simulink model "ASM_Traffic_A11"  (R2026a)
settings: Solver=ode1  StartTime=SIM.tstart.v  StopTime=SIM.tend.v  FixedStep=SIM.StepSize.v
PostLoadFcn:
  | if any(exist('dsrtsu_mdlpostloadfcn', 'file') ~= 0), dsrtsu_mdlpostloadfcn('Execute', bdroot); end
  | try, asm_mdl_postloadfcn(bdroot, 'UpdateModel', 3600); catch, disp(lasterr); end,
InitFcn:
  | , if any(exist('rtifpga_mdlclblib', 'file') ~= 0), rtifpga_mdlclblib('Init', bdroot); end,
  | , if any(exist('dsmpb_private', 'file') ~= 0), dsmpb_private('dsmpb_mdlclblib', 'Init', bdroot); end,
undefined symbols (not defined in the file): _to_, a0b2, ASM_BrakeHydraulics_DemoSystems, ASM_VehicleDynamics_DemoSystems, b98103fe8ad365046cd0, BrakeCircuit, controllerConfig, CPT, Crankshaft, DiscIntNeverNeededParam, dsmsi, FinalDriveAssembly, instance, MDL, ModeSignals, mu, Pos_BrakePedal_Maneuver, rad, RefSignals, s_to_rpm, SIM, SoftECU, Suspension, Tire, Transmission
libraries: ASM_Traffic_lib x135, simulink x98, ASM_Utils_lib x77, ASM_VehicleDynamics_lib x70, ASM_Environment_lib x22, dsmpblib x20, dsmsilib x15, MDLD_Utils_lib x10, ASM_BrakeHydraulics_lib x3, sl_discontinuities x2
(part 29 of 63)

== system ASM_Traffic_A11/VehicleDynamics/Control/Sw_ECU_Brake_Signals/Enable_TrqDecrease_Fast_ESP[0|1] ==
  SoftECU : Inport
  RealECU : Inport  Port=2
  Const_Enable_TrqDecrease_Fast[0|1] : Constant  Value=0
  MultiPortSwitch : MultiPortSwitch
  Sw_Enable_TrqDecrease_Fast[1SoftECU|2RealECU|3Const] : Constant  Value=CPT.MDL_SW.Sw_Enable_TrqDecrease_Fast_ESP.v
  Enable_TrqDecrease_Fast[0|1] : Outport  VectorParamsAs1DForOutWhenUnconnected=off
  wires:
  Sw_Enable_TrqDecrease_Fast[1SoftECU|2RealECU|3Const]/1 -> MultiPortSwitch/1
  SoftECU/1 -> MultiPortSwitch/2
  RealECU/1 -> MultiPortSwitch/3
  Const_Enable_TrqDecrease_Fast[0|1]/1 -> MultiPortSwitch/4
  MultiPortSwitch/1 -> Enable_TrqDecrease_Fast[0|1]/1

== system ASM_Traffic_A11/VehicleDynamics/Control/Sw_ECU_Brake_Signals/Enable_TrqDecrease_Slow_ESP[0|1] ==
  SoftECU : Inport
  RealECU : Inport  Port=2
  Const_Enable_TrqDecrease_Slow[0|1] : Constant  Value=0
  MultiPortSwitch : MultiPortSwitch
  Sw_Enable_TrqDecrease_Slow[1SoftECU|2RealECU|3Const] : Constant  Value=CPT.MDL_SW.Sw_Enable_TrqDecrease_Slow_ESP.v
  Enable_TrqDecrease_Slow[0|1] : Outport  VectorParamsAs1DForOutWhenUnconnected=off
  wires:
  Sw_Enable_TrqDecrease_Slow[1SoftECU|2RealECU|3Const]/1 -> MultiPortSwitch/1
  SoftECU/1 -> MultiPortSwitch/2
  RealECU/1 -> MultiPortSwitch/3
  Const_Enable_TrqDecrease_Slow[0|1]/1 -> MultiPortSwitch/4
  MultiPortSwitch/1 -> Enable_TrqDecrease_Slow[0|1]/1

== system ASM_Traffic_A11/VehicleDynamics/Control/Sw_ECU_Brake_Signals/Enable_TrqIncrease_ESP[0|1] ==
  SoftECU : Inport
  RealECU : Inport  Port=2
  Const_Enable_TrqIncrease[0|1] : Constant  Value=0
  MultiPortSwitch : MultiPortSwitch
  Sw_Enable_TrqIncrease[1SoftECU|2RealECU|3Const] : Constant  Value=CPT.MDL_SW.Sw_Enable_TrqIncrease_ESP.v
  Enable_TrqIncrease[0|1] : Outport  VectorParamsAs1DForOutWhenUnconnected=off
  wires:
  Sw_Enable_TrqIncrease[1SoftECU|2RealECU|3Const]/1 -> MultiPortSwitch/1
  SoftECU/1 -> MultiPortSwitch/2
  RealECU/1 -> MultiPortSwitch/3
  Const_Enable_TrqIncrease[0|1]/1 -> MultiPortSwitch/4
  MultiPortSwitch/1 -> Enable_TrqIncrease[0|1]/1

== system ASM_Traffic_A11/VehicleDynamics/Control/Sw_ECU_Brake_Signals/Enable_p_Brake_Desired[0|1] ==
  SoftECU : Inport
  RealECU : Inport  Port=2
  Const_Enable_p_Brake_Desired[0|1] : Constant  Value=0
  MultiPortSwitch : MultiPortSwitch
  Sw_Enable_p_Brake_Desired[1SoftECU|2RealECU|3Const] : Constant  Value=CPT.MDL_SW.Sw_Enable_p_Brake_Desired.v
  Enable_p_Brake_Desired[0|1] : Outport  VectorParamsAs1DForOutWhenUnconnected=off
  wires:
  MultiPortSwitch/1 -> Enable_p_Brake_Desired[0|1]/1
  Const_Enable_p_Brake_Desired[0|1]/1 -> MultiPortSwitch/4
  RealECU/1 -> MultiPortSwitch/3
  SoftECU/1 -> MultiPortSwitch/2
  Sw_Enable_p_Brake_Desired[1SoftECU|2RealECU|3Const]/1 -> MultiPortSwitch/1

== system ASM_Traffic_A11/VehicleDynamics/Control/Sw_ECU_Brake_Signals/Trq_DecreaseRequest_Fast_ESP[Nm] ==
  SoftECU : Inport
  RealECU : Inport  Port=2
  Const_Trq_DecreaseRequest_Fast[Nm] : Constant  Value=0
  MultiPortSwitch : MultiPortSwitch
  Sw_Trq_DecreaseRequest_Fast[1SoftECU|2RealECU|3Const] : Constant  Value=CPT.MDL_SW.Sw_Trq_DecreaseRequest_Fast_ESP.v
  Trq_DecreaseRequest_Fast[Nm] : Outport  VectorParamsAs1DForOutWhenUnconnected=off
  wires:
  MultiPortSwitch/1 -> Trq_DecreaseRequest_Fast[Nm]/1
  Const_Trq_DecreaseRequest_Fast[Nm]/1 -> MultiPortSwitch/4
  RealECU/1 -> MultiPortSwitch/3
  SoftECU/1 -> MultiPortSwitch/2
  Sw_Trq_DecreaseRequest_Fast[1SoftECU|2RealECU|3Const]/1 -> MultiPortSwitch/1

== system ASM_Traffic_A11/VehicleDynamics/Control/Sw_ECU_Brake_Signals/Trq_DecreaseRequest_Slow_ESP[Nm] ==
  SoftECU : Inport
  RealECU : Inport  Port=2
  Const_Trq_DecreaseRequest_Slow[Nm] : Constant  Value=0
  MultiPortSwitch : MultiPortSwitch
  Sw_Trq_DecreaseRequest_Slow[1SoftECU|2RealECU|3Const] : Constant  Value=CPT.MDL_SW.Sw_Trq_DecreaseRequest_Slow_ESP.v
  Trq_DecreaseRequest_Slow[Nm] : Outport  VectorParamsAs1DForOutWhenUnconnected=off
  wires:
  MultiPortSwitch/1 -> Trq_DecreaseRequest_Slow[Nm]/1
  Const_Trq_DecreaseRequest_Slow[Nm]/1 -> MultiPortSwitch/4
  RealECU/1 -> MultiPortSwitch/3
  SoftECU/1 -> MultiPortSwitch/2
  Sw_Trq_DecreaseRequest_Slow[1SoftECU|2RealECU|3Const]/1 -> MultiPortSwitch/1

== system ASM_Traffic_A11/VehicleDynamics/Control/Sw_ECU_Brake_Signals/Trq_IncreaseRequest_ESP[Nm] ==
  SoftECU : Inport
  RealECU : Inport  Port=2
  Const_Trq_IncreaseRequest[Nm] : Constant  Value=0
  MultiPortSwitch : MultiPortSwitch
  Sw_Trq_IncreaseRequest[1SoftECU|2RealECU|3Const] : Constant  Value=CPT.MDL_SW.Sw_Trq_IncreaseRequest_ESP.v
  Trq_IncreaseRequest[Nm] : Outport  VectorParamsAs1DForOutWhenUnconnected=off
  wires:
  MultiPortSwitch/1 -> Trq_IncreaseRequest[Nm]/1
  Const_Trq_IncreaseRequest[Nm]/1 -> MultiPortSwitch/4
  RealECU/1 -> MultiPortSwitch/3
  SoftECU/1 -> MultiPortSwitch/2
  Sw_Trq_IncreaseRequest[1SoftECU|2RealECU|3Const]/1 -> MultiPortSwitch/1

== system ASM_Traffic_A11/VehicleDynamics/Control/Sw_ECU_Brake_Signals/p_Brake_Desired[bar] ==
  SoftECU : Inport
  RealECU : Inport  Port=2
  Const_p_Brake_Desired[bar] : Constant  Value=0
  MultiPortSwitch : MultiPortSwitch
  Sw_p_Brake_Desired[1SoftECU|2RealECU|3Const] : Constant  Value=CPT.MDL_SW.Sw_p_Brake_Desired.v
  p_Brake_Desired[bar] : Outport  VectorParamsAs1DForOutWhenUnconnected=off
  wires:
  Sw_p_Brake_Desired[1SoftECU|2RealECU|3Const]/1 -> MultiPortSwitch/1
  SoftECU/1 -> MultiPortSwitch/2
  RealECU/1 -> MultiPortSwitch/3
  Const_p_Brake_Desired[bar]/1 -> MultiPortSwitch/4
  MultiPortSwitch/1 -> p_Brake_Desired[bar]/1

== system ASM_Traffic_A11/VehicleDynamics/Control/Sw_ECU_Steering_Signals/Trq_PowerSteering[Nm] ==
  SoftECU : Inport
  RealECU : Inport  Port=2
  Const_Trq_PowerSteering[Nm] : Constant  Value=0
  MultiPortSwitch : MultiPortSwitch
  Sw_PowerSteering[1SoftECU|2RealECU|3Const] : Constant  Value=CPT.MDL_SW.Sw_PowerSteering.v
  Trq_PowerSteering[Nm] : Outport  VectorParamsAs1DForOutWhenUnconnected=off
  wires:
  MultiPortSwitch/1 -> Trq_PowerSteering[Nm]/1
  Const_Trq_PowerSteering[Nm]/1 -> MultiPortSwitch/4
  RealECU/1 -> MultiPortSwitch/3
  SoftECU/1 -> MultiPortSwitch/2
  Sw_PowerSteering[1SoftECU|2RealECU|3Const]/1 -> MultiPortSwitch/1

== system ASM_Traffic_A11/VehicleDynamics/Control/UserInterface/ASMSignalBus_Control ==
  In : Inport
  Terminator_1 : Terminator
  tag scope: ASMBUS_VehicleDynamics_Control=global
  wires:
  In/1 -> [ASMBUS_VehicleDynamics_Control]  "Control"
  [ASMBUS_VehicleDynamics_Control] -> Terminator_1/1

== system ASM_Traffic_A11/VehicleDynamics/Control/UserInterface/DISP_Control ==
  In : Inport
  ECU_Brake : Subsystem
  wires:
  In/1 -> ECU_Brake/1(In)

== system ASM_Traffic_A11/VehicleDynamics/Control/UserInterface/PAR_Control ==
  ECU_Brake : Subsystem
  Out : Outport  VectorParamsAs1DForOutWhenUnconnected=off
  wires:
  ECU_Brake/1(SoftECU_Brake) -> Out/1

== system ASM_Traffic_A11/VehicleDynamics/Interface_In/ExternalSignals/ExternalECU_Brake ==
  Enable_p_Brake_Desired[0|1] : Inport
  p_Brake_Desired[bar] : Inport  Port=2
  Enable_TrqDecrease_Fast_ESP[0|1] : Inport  Port=3
  Trq_DecreaseRequest_Fast_ESP[Nm] : Inport  Port=4
  Enable_TrqDecrease_Slow_ESP[0|1] : Inport  Port=5
  Trq_DecreaseRequest_Slow_ESP[Nm] : Inport  Port=6
  Enable_TrqIncrease_ESP[0|1] : Inport  Port=7
  Trq_IncreaseRequest_ESP[Nm] : Inport  Port=8
  ECU_ESP_Mode[0None|1ABS|2ESP|3ASR] : Inport  Port=9
  Ctrl_InletValve_FL[0_1] : Inport  Port=10
  Ctrl_InletValve_FR[0_1] : Inport  Port=11
  Ctrl_InletValve_RL[0_1] : Inport  Port=12
  Ctrl_InletValve_RR[0_1] : Inport  Port=13
  Ctrl_OutletValve_FL[0_1] : Inport  Port=14
  Ctrl_OutletValve_FR[0_1] : Inport  Port=15
  Ctrl_OutletValve_RL[0_1] : Inport  Port=16
  Ctrl_OutletValve_RR[0_1] : Inport  Port=17
  Ctrl_PreChargeValve_1[0_1] : Inport  Port=18
  Ctrl_PreChargeValve_2[0_1] : Inport  Port=19
  Ctrl_ChangeOverValve_1[0_1] : Inport  Port=20
  Ctrl_ChangeOverValve_2[0_1] : Inport  Port=21
  Ctrl_HydPump[0_1] : Inport  Port=22
  Bus Creator2 : BusCreator  Inputs=22
  Out : Outport  VectorParamsAs1DForOutWhenUnconnected=off
  wires:
  Ctrl_InletValve_FL[0_1]/1 -> Bus Creator2/10  "Ctrl_InletValve_FL[0_1]"
  Bus Creator2/1 -> Out/1  "Brake"
  Ctrl_InletValve_FR[0_1]/1 -> Bus Creator2/11  "Ctrl_InletValve_FR[0_1]"
  Ctrl_InletValve_RL[0_1]/1 -> Bus Creator2/12  "Ctrl_InletValve_RL[0_1]"
  Ctrl_InletValve_RR[0_1]/1 -> Bus Creator2/13  "Ctrl_InletValve_RR[0_1]"
  Ctrl_OutletValve_FL[0_1]/1 -> Bus Creator2/14  "Ctrl_OutletValve_FL[0_1]"
  Ctrl_OutletValve_FR[0_1]/1 -> Bus Creator2/15  "Ctrl_OutletValve_FR[0_1]"
  Ctrl_OutletValve_RL[0_1]/1 -> Bus Creator2/16  "Ctrl_OutletValve_RL[0_1]"
  Ctrl_OutletValve_RR[0_1]/1 -> Bus Creator2/17  "Ctrl_OutletValve_RR[0_1]"
  Ctrl_PreChargeValve_1[0_1]/1 -> Bus Creator2/18  "Ctrl_PreChargeValve_1[0_1]"
  Ctrl_PreChargeValve_2[0_1]/1 -> Bus Creator2/19  "Ctrl_PreChargeValve_2[0_1]"
  Ctrl_ChangeOverValve_1[0_1]/1 -> Bus Creator2/20  "Ctrl_ChangeOverValve_1[0_1]"
  Ctrl_ChangeOverValve_2[0_1]/1 -> Bus Creator2/21  "Ctrl_ChangeOverValve_2[0_1]"
  Ctrl_HydPump[0_1]/1 -> Bus Creator2/22  "Ctrl_HydPump[0_1]"
  Enable_TrqDecrease_Fast_ESP[0|1]/1 -> Bus Creator2/3  "Enable_TrqDecrease_Fast_ESP[0|1]"
  Trq_DecreaseRequest_Slow_ESP[Nm]/1 -> Bus Creator2/6  "Trq_DecreaseRequest_Slow_ESP[Nm]"
  Enable_TrqIncrease_ESP[0|1]/1 -> Bus Creator2/7  "Enable_TrqIncrease_ESP[0|1]"
  Trq_IncreaseRequest_ESP[Nm]/1 -> Bus Creator2/8  "Trq_IncreaseRequest_ESP[Nm]"
  Trq_DecreaseRequest_Fast_ESP[Nm]/1 -> Bus Creator2/4  "Trq_DecreaseRequest_Fast_ESP[Nm]"
  Enable_TrqDecrease_Slow_ESP[0|1]/1 -> Bus Creator2/5  "Enable_TrqDecrease_Slow_ESP[0|1]"
  Enable_p_Brake_Desired[0|1]/1 -> Bus Creator2/1  "Enable_p_Brake_Desired[0|1]"
  p_Brake_Desired[bar]/1 -> Bus Creator2/2  "p_Brake_Desired[bar]"
  ECU_ESP_Mode[0None|1ABS|2ESP|3ASR]/1 -> Bus Creator2/9  "ECU_ESP_Mode[0None|1ABS|2ESP|3ASR]"

== system ASM_Traffic_A11/VehicleDynamics/Interface_In/ExternalSignals/ExternalECU_Steering ==
  Trq_PowerSteering[Nm] : Inport
  Bus Creator6 : BusCreator  Inputs=1
  Out : Outport  VectorParamsAs1DForOutWhenUnconnected=off
  wires:
  Bus Creator6/1 -> Out/1  "Steering"
  Trq_PowerSteering[Nm]/1 -> Bus Creator6/1  "Trq_PowerSteering[Nm]"

== system ASM_Traffic_A11/VehicleDynamics/Interface_In/ExternalSignals/ExternalPlant_EPSMotor ==
  Angle_EPSMotor[rad] : Inport
  Angle_dt_EPSMotor[rad|s] : Inport  Port=2
  Bus Creator6 : BusCreator  Inputs=2
  Out : Outport  VectorParamsAs1DForOutWhenUnconnected=off
  wires:
  Angle_dt_EPSMotor[rad|s]/1 -> Bus Creator6/2  "Angle_dt_EPSMotor[rad|s]"
  Bus Creator6/1 -> Out/1  "EPSMotor"
  Angle_EPSMotor[rad]/1 -> Bus Creator6/1  "Angle_EPSMotor[rad]"

== system ASM_Traffic_A11/VehicleDynamics/Interface_In/ExternalSignals/ExternalPlant_RollerDyno ==
  Angle_Gamma_FL_Wheel[deg] : Inport
  omega_Wheel[FL;FR;RL;RR][rad|s] : Inport  Port=2
  Bus Creator6 : BusCreator  Inputs=2
  Out : Outport  VectorParamsAs1DForOutWhenUnconnected=off
  wires:
  Angle_Gamma_FL_Wheel[deg]/1 -> Bus Creator6/1  "Angle_Gamma_FL_Wheel[deg]"
  omega_Wheel[FL;FR;RL;RR][rad|s]/1 -> Bus Creator6/2  "omega_Wheel[FL;FR;RL;RR][rad|s]"
  Bus Creator6/1 -> Out/1  "RollerDyno"

== system ASM_Traffic_A11/VehicleDynamics/Interface_In/ExternalSignals/ExternalPlant_Steering ==
  Displ_Steering[m] : Inport
  Displ_Steering_dt[m|s] : Inport  Port=2
  Bus Creator6 : BusCreator  Inputs=2
  Out : Outport  VectorParamsAs1DForOutWhenUnconnected=off
  wires:
  Displ_Steering_dt[m|s]/1 -> Bus Creator6/2  "Displ_Steering_dt[m|s]"
  Displ_Steering[m]/1 -> Bus Creator6/1  "Displ_Steering[m]"
  Bus Creator6/1 -> Out/1  "Steering"

== system ASM_Traffic_A11/VehicleDynamics/Interface_In/ModelSignals/Angle_SteeringWheel[deg]_ ==
  In1 : Inport
  Gain : Gain  SaturateOnIntegerOverflow=on  OutDataTypeStr=Inherit: Same as input  ParamDataTypeStr=Inherit: Same as input
  Out1 : Outport  VectorParamsAs1DForOutWhenUnconnected=off
  wires:
  In1/1 -> Gain/1
  Gain/1 -> Out1/1

== system ASM_Traffic_A11/VehicleDynamics/Interface_In/ModelSignals/Angle_Vehicle_Init_CoorSys_E[x;y;z][rad]_ ==
  In1 : Inport
  Gain : Gain  SaturateOnIntegerOverflow=on  OutDataTypeStr=Inherit: Same as input  ParamDataTypeStr=Inherit: Same as input
  Out1 : Outport  VectorParamsAs1DForOutWhenUnconnected=off
  wires:
  In1/1 -> Gain/1
  Gain/1 -> Out1/1

== system ASM_Traffic_A11/VehicleDynamics/Interface_In/ModelSignals/Const_Steering_Mode_Manual[1Angle|2Trq]_ ==
  In1 : Inport
  Gain : Gain  SaturateOnIntegerOverflow=on  OutDataTypeStr=Inherit: Same as input  ParamDataTypeStr=Inherit: Same as input
  Out1 : Outport  VectorParamsAs1DForOutWhenUnconnected=off
  wires:
  Gain/1 -> Out1/1
  In1/1 -> Gain/1

== system ASM_Traffic_A11/VehicleDynamics/Interface_In/ModelSignals/ECU_Commands[]_ ==
  In1 : Inport
  Gain : Gain  SaturateOnIntegerOverflow=on  OutDataTypeStr=Inherit: Same as input  ParamDataTypeStr=Inherit: Same as input
  Out1 : Outport  VectorParamsAs1DForOutWhenUnconnected=off
  wires:
  In1/1 -> Gain/1
  Gain/1 -> Out1/1

== system ASM_Traffic_A11/VehicleDynamics/Interface_In/ModelSignals/Enable_Trq_Brake_Extern[0|1]_ ==
  In1 : Inport
  Gain : Gain  SaturateOnIntegerOverflow=on  OutDataTypeStr=Inherit: Same as input  ParamDataTypeStr=Inherit: Same as input
  Out1 : Outport  VectorParamsAs1DForOutWhenUnconnected=off
  wires:
  In1/1 -> Gain/1
  Gain/1 -> Out1/1

== system ASM_Traffic_A11/VehicleDynamics/Interface_In/ModelSignals/Fric_Coeff_CP[FL;FR;RL;RR][]_ ==
  In1 : Inport
  Gain : Gain  SaturateOnIntegerOverflow=on  OutDataTypeStr=Inherit: Same as input  ParamDataTypeStr=Inherit: Same as input
  Out1 : Outport  VectorParamsAs1DForOutWhenUnconnected=off
  wires:
  In1/1 -> Gain/1
  Gain/1 -> Out1/1

== system ASM_Traffic_A11/VehicleDynamics/Interface_In/ModelSignals/Keep_VehiclePosition[0|1]_ ==
  In1 : Inport
  Gain : Gain  SaturateOnIntegerOverflow=on  OutDataTypeStr=Inherit: Same as input  ParamDataTypeStr=Inherit: Same as input
  Out1 : Outport  VectorParamsAs1DForOutWhenUnconnected=off
  wires:
  In1/1 -> Gain/1
  Gain/1 -> Out1/1

== system ASM_Traffic_A11/VehicleDynamics/Interface_In/ModelSignals/M_Articulated_T[1x36]_ ==
  In1 : Inport
  Gain : Gain  SaturateOnIntegerOverflow=on  OutDataTypeStr=Inherit: Same as input  ParamDataTypeStr=Inherit: Same as input
  Out1 : Outport  VectorParamsAs1DForOutWhenUnconnected=off
  wires:
  In1/1 -> Gain/1
  Gain/1 -> Out1/1

== system ASM_Traffic_A11/VehicleDynamics/Interface_In/ModelSignals/Pos_AccPedal[%]_ ==
  In1 : Inport
  Gain : Gain  SaturateOnIntegerOverflow=on  OutDataTypeStr=Inherit: Same as input  ParamDataTypeStr=Inherit: Same as input
  Out1 : Outport  VectorParamsAs1DForOutWhenUnconnected=off
  wires:
  In1/1 -> Gain/1
  Gain/1 -> Out1/1

== system ASM_Traffic_A11/VehicleDynamics/Interface_In/ModelSignals/Pos_BrakePedal[%]_ ==
  In1 : Inport
  Gain : Gain  SaturateOnIntegerOverflow=on  OutDataTypeStr=Inherit: Same as input  ParamDataTypeStr=Inherit: Same as input
  Out1 : Outport  VectorParamsAs1DForOutWhenUnconnected=off
  wires:
  In1/1 -> Gain/1
  Gain/1 -> Out1/1

== system ASM_Traffic_A11/VehicleDynamics/Interface_In/ModelSignals/Pos_Vehicle_Init_CoorSys_E[x;y;z][m]_ ==
  In1 : Inport
  Gain : Gain  SaturateOnIntegerOverflow=on  OutDataTypeStr=Inherit: Same as input  ParamDataTypeStr=Inherit: Same as input
  Out1 : Outport  VectorParamsAs1DForOutWhenUnconnected=off
  wires:
  In1/1 -> Gain/1
  Gain/1 -> Out1/1

== system ASM_Traffic_A11/VehicleDynamics/Interface_In/ModelSignals/Pos_z_CP[FL;FR;RL;RR][m]_ ==
  In1 : Inport
  Gain : Gain  SaturateOnIntegerOverflow=on  OutDataTypeStr=Inherit: Same as input  ParamDataTypeStr=Inherit: Same as input
  Out1 : Outport  VectorParamsAs1DForOutWhenUnconnected=off
  wires:
  In1/1 -> Gain/1
  Gain/1 -> Out1/1

== system ASM_Traffic_A11/VehicleDynamics/Interface_In/ModelSignals/Q_Articulated_T[6x1]_ ==
  In1 : Inport
  Gain : Gain  SaturateOnIntegerOverflow=on  OutDataTypeStr=Inherit: Same as input  ParamDataTypeStr=Inherit: Same as input
  Out1 : Outport  VectorParamsAs1DForOutWhenUnconnected=off
  wires:
  In1/1 -> Gain/1
  Gain/1 -> Out1/1

== system ASM_Traffic_A11/VehicleDynamics/Interface_In/ModelSignals/Reset_VehicleStates[0|1]_ ==
  In1 : Inport
  Gain : Gain  SaturateOnIntegerOverflow=on  OutDataTypeStr=Inherit: Same as input  ParamDataTypeStr=Inherit: Same as input
  Out1 : Outport  VectorParamsAs1DForOutWhenUnconnected=off
  wires:
  In1/1 -> Gain/1
  Gain/1 -> Out1/1

== system ASM_Traffic_A11/VehicleDynamics/Interface_In/ModelSignals/Sw_Ignition[0Off|1On]_ ==
  In1 : Inport
  Gain : Gain  SaturateOnIntegerOverflow=on  OutDataTypeStr=Inherit: Same as input  ParamDataTypeStr=Inherit: Same as input
  Out1 : Outport  VectorParamsAs1DForOutWhenUnconnected=off
  wires:
  In1/1 -> Gain/1
  Gain/1 -> Out1/1

== system ASM_Traffic_A11/VehicleDynamics/Interface_In/ModelSignals/Sw_ModelDeskPlottingInterface[0Disabled|1Enabled]_ ==
  In1 : Inport
  Gain : Gain
  Out1 : Outport
  wires:
  Gain/1 -> Out1/1
  In1/1 -> Gain/1

== system ASM_Traffic_A11/VehicleDynamics/Interface_In/ModelSignals/Sw_ModelPortBlocks[0Disabled|1Enabled]_ ==
  In1 : Inport
  Gain : Gain
  Out1 : Outport
  wires:
  Gain/1 -> Out1/1
  In1/1 -> Gain/1

== system ASM_Traffic_A11/VehicleDynamics/Interface_In/ModelSignals/Sw_ParkingBrake[0Off|1On]_ ==
  In1 : Inport
  Gain : Gain  SaturateOnIntegerOverflow=on  OutDataTypeStr=Inherit: Same as input  ParamDataTypeStr=Inherit: Same as input
  Out1 : Outport  VectorParamsAs1DForOutWhenUnconnected=off
  wires:
  In1/1 -> Gain/1
  Gain/1 -> Out1/1

== system ASM_Traffic_A11/VehicleDynamics/Interface_In/ModelSignals/Sw_SteeringMode[1Angle|2Trq]_ ==
  In1 : Inport
  Gain : Gain  SaturateOnIntegerOverflow=on  OutDataTypeStr=Inherit: Same as input  ParamDataTypeStr=Inherit: Same as input
  Out1 : Outport  VectorParamsAs1DForOutWhenUnconnected=off
  wires:
  In1/1 -> Gain/1
  Gain/1 -> Out1/1

== system ASM_Traffic_A11/VehicleDynamics/Interface_In/ModelSignals/Sw_Steering_Mode[1Manual|2ManSched]_ ==
  In1 : Inport
  Gain : Gain  SaturateOnIntegerOverflow=on  OutDataTypeStr=Inherit: Same as input  ParamDataTypeStr=Inherit: Same as input
  Out1 : Outport  VectorParamsAs1DForOutWhenUnconnected=off
  wires:
  Gain/1 -> Out1/1
  In1/1 -> Gain/1

== system ASM_Traffic_A11/VehicleDynamics/Interface_In/ModelSignals/Sw_Tire_Parameter_Set_CP[FL;FR;RL;RR][1|2|3|4]_ ==
  In1 : Inport
  Gain : Gain  SaturateOnIntegerOverflow=on  OutDataTypeStr=Inherit: Same as input  ParamDataTypeStr=Inherit: Same as input
  Out1 : Outport  VectorParamsAs1DForOutWhenUnconnected=off
  wires:
  In1/1 -> Gain/1
  Gain/1 -> Out1/1

== system ASM_Traffic_A11/VehicleDynamics/Interface_In/ModelSignals/T_Ambient[degC]_ ==
  In1 : Inport
  Gain : Gain  SaturateOnIntegerOverflow=on  OutDataTypeStr=Inherit: Same as input  ParamDataTypeStr=Inherit: Same as input
  Out1 : Outport  VectorParamsAs1DForOutWhenUnconnected=off
  wires:
  In1/1 -> Gain/1
  Gain/1 -> Out1/1

== system ASM_Traffic_A11/VehicleDynamics/Interface_In/ModelSignals/Trq_Brake_Request_Extern[Nm]_ ==
  In1 : Inport
  Gain : Gain  SaturateOnIntegerOverflow=on  OutDataTypeStr=Inherit: Same as input  ParamDataTypeStr=Inherit: Same as input
  Out1 : Outport  VectorParamsAs1DForOutWhenUnconnected=off
  wires:
  In1/1 -> Gain/1
  Gain/1 -> Out1/1

== system ASM_Traffic_A11/VehicleDynamics/Interface_In/ModelSignals/Trq_Driver_External[Nm]_ ==
  In1 : Inport
  Gain : Gain  SaturateOnIntegerOverflow=on  OutDataTypeStr=Inherit: Same as input  ParamDataTypeStr=Inherit: Same as input
  Out1 : Outport  VectorParamsAs1DForOutWhenUnconnected=off
  wires:
  In1/1 -> Gain/1
  Gain/1 -> Out1/1

== system ASM_Traffic_A11/VehicleDynamics/Interface_In/ModelSignals/Trq_EM_Front[Nm]_ ==
  In1 : Inport
  Gain : Gain  SaturateOnIntegerOverflow=on  OutDataTypeStr=Inherit: Same as input  ParamDataTypeStr=Inherit: Same as input
  Out1 : Outport  VectorParamsAs1DForOutWhenUnconnected=off
  wires:
  Gain/1 -> Out1/1
  In1/1 -> Gain/1

== system ASM_Traffic_A11/VehicleDynamics/Interface_In/ModelSignals/Trq_Eff_Engine[Nm]_ ==
  In1 : Inport
  Gain : Gain  SaturateOnIntegerOverflow=on  OutDataTypeStr=Inherit: Same as input  ParamDataTypeStr=Inherit: Same as input
  Out1 : Outport  VectorParamsAs1DForOutWhenUnconnected=off
  wires:
  In1/1 -> Gain/1
  Gain/1 -> Out1/1

== system ASM_Traffic_A11/VehicleDynamics/Interface_In/ModelSignals/Trq_Hitch_CoorSys_V[x;y;z][Nm]_ ==
  In1 : Inport
  Gain : Gain  SaturateOnIntegerOverflow=on  OutDataTypeStr=Inherit: Same as input  ParamDataTypeStr=Inherit: Same as input
  Out1 : Outport  VectorParamsAs1DForOutWhenUnconnected=off
  wires:
  In1/1 -> Gain/1
  Gain/1 -> Out1/1

== system ASM_Traffic_A11/VehicleDynamics/Interface_In/ModelSignals/Trq_Request_Brake[Nm]_ ==
  In1 : Inport
  Gain : Gain  SaturateOnIntegerOverflow=on  OutDataTypeStr=Inherit: Same as input  ParamDataTypeStr=Inherit: Same as input
  Out1 : Outport  VectorParamsAs1DForOutWhenUnconnected=off
  wires:
  Gain/1 -> Out1/1
  In1/1 -> Gain/1

== system ASM_Traffic_A11/VehicleDynamics/Interface_In/ModelSignals/Trq_Shaft[FL,FR,RL,RR][Nm]_ ==
  In1 : Inport
  Gain : Gain  SaturateOnIntegerOverflow=on  OutDataTypeStr=Inherit: Same as input  ParamDataTypeStr=Inherit: Same as input
  Out1 : Outport  VectorParamsAs1DForOutWhenUnconnected=off
  wires:
  In1/1 -> Gain/1
  Gain/1 -> Out1/1

== system ASM_Traffic_A11/VehicleDynamics/Interface_In/ModelSignals/UnitVec_z_CP[FL;FR;RL;RR][x;y;z]_ ==
  In1 : Inport
  Gain : Gain  SaturateOnIntegerOverflow=on  OutDataTypeStr=Inherit: Same as input  ParamDataTypeStr=Inherit: Same as input
  Out1 : Outport  VectorParamsAs1DForOutWhenUnconnected=off
  wires:
  In1/1 -> Gain/1
  Gain/1 -> Out1/1

== system ASM_Traffic_A11/VehicleDynamics/Interface_In/ModelSignals/Vehicle_Topology[-2|-1|0|2]_ ==
  In1 : Inport
  Gain : Gain  SaturateOnIntegerOverflow=on  OutDataTypeStr=Inherit: Same as input  ParamDataTypeStr=Inherit: Same as input
  Out1 : Outport  VectorParamsAs1DForOutWhenUnconnected=off
  wires:
  In1/1 -> Gain/1
  Gain/1 -> Out1/1

== system ASM_Traffic_A11/VehicleDynamics/Interface_In/ModelSignals/p_Ambient[Pa]_ ==
  In1 : Inport
  Gain : Gain  SaturateOnIntegerOverflow=on  OutDataTypeStr=Inherit: Same as input  ParamDataTypeStr=Inherit: Same as input
  Out1 : Outport  VectorParamsAs1DForOutWhenUnconnected=off
  wires:
  In1/1 -> Gain/1
  Gain/1 -> Out1/1

== system ASM_Traffic_A11/VehicleDynamics/Interface_In/ModelSignals/q_dt_Vehicle_Init[6x1]_ ==
  In1 : Inport
  Gain : Gain  SaturateOnIntegerOverflow=on  OutDataTypeStr=Inherit: Same as input  ParamDataTypeStr=Inherit: Same as input
  Out1 : Outport  VectorParamsAs1DForOutWhenUnconnected=off
  wires:
  In1/1 -> Gain/1
  Gain/1 -> Out1/1

== system ASM_Traffic_A11/VehicleDynamics/Interface_In/ModelSignals/v_Wind_Coor_Sys_E[x;y;z][m|s]_ ==
  In1 : Inport
  Gain : Gain  SaturateOnIntegerOverflow=on  OutDataTypeStr=Inherit: Same as input  ParamDataTypeStr=Inherit: Same as input
  Out1 : Outport  VectorParamsAs1DForOutWhenUnconnected=off
  wires:
  In1/1 -> Gain/1
  Gain/1 -> Out1/1

== system ASM_Traffic_A11/VehicleDynamics/Interface_Out/Animation/Angle_FL_Wheel[Toe;Camber][deg] ==
  In1 : Inport
  Out1 : Outport  VectorParamsAs1DForOutWhenUnconnected=off
  wires:
  In1/1 -> Out1/1

== system ASM_Traffic_A11/VehicleDynamics/Interface_Out/Animation/Angle_FR_Wheel[Toe;Camber][deg] ==
  In1 : Inport
  Out1 : Outport  VectorParamsAs1DForOutWhenUnconnected=off
  wires:
  In1/1 -> Out1/1

== system ASM_Traffic_A11/VehicleDynamics/Interface_Out/Animation/Angle_RL_Wheel[Toe;Camber][deg] ==
  In1 : Inport
  Out1 : Outport  VectorParamsAs1DForOutWhenUnconnected=off
  wires:
  In1/1 -> Out1/1

== system ASM_Traffic_A11/VehicleDynamics/Interface_Out/Animation/Angle_RR_Wheel[Toe;Camber][deg] ==
  In1 : Inport
  Out1 : Outport  VectorParamsAs1DForOutWhenUnconnected=off
  wires:
  In1/1 -> Out1/1

== system ASM_Traffic_A11/VehicleDynamics/Interface_Out/Animation/Angle_Rot_FL_Wheel[deg] ==
  In1 : Inport
  Out1 : Outport  VectorParamsAs1DForOutWhenUnconnected=off
  wires:
  In1/1 -> Out1/1

== system ASM_Traffic_A11/VehicleDynamics/Interface_Out/Animation/Angle_Rot_FR_Wheel[deg] ==
  In1 : Inport
  Out1 : Outport  VectorParamsAs1DForOutWhenUnconnected=off
  wires:
  In1/1 -> Out1/1

== system ASM_Traffic_A11/VehicleDynamics/Interface_Out/Animation/Angle_Rot_RL_Wheel[deg] ==
  In1 : Inport
  Out1 : Outport  VectorParamsAs1DForOutWhenUnconnected=off
  wires:
  In1/1 -> Out1/1

== system ASM_Traffic_A11/VehicleDynamics/Interface_Out/Animation/Angle_Rot_RR_Wheel[deg] ==
  In1 : Inport
  Out1 : Outport  VectorParamsAs1DForOutWhenUnconnected=off
  wires:
  In1/1 -> Out1/1

== system ASM_Traffic_A11/VehicleDynamics/Interface_Out/Animation/Angle_SteeringWheel[deg] ==
  In1 : Inport
  Out1 : Outport  VectorParamsAs1DForOutWhenUnconnected=off
  wires:
  In1/1 -> Out1/1

== system ASM_Traffic_A11/VehicleDynamics/Interface_Out/Animation/Angle_Vehicle_CoorSys_E[x;y;z][deg] ==
  In1 : Inport
  Out1 : Outport  VectorParamsAs1DForOutWhenUnconnected=off
  wires:
  In1/1 -> Out1/1

== system ASM_Traffic_A11/VehicleDynamics/Interface_Out/Animation/Angle_Yaw_Vehicle_CoorSys_E[deg] ==
  In1 : Inport
  Out1 : Outport  VectorParamsAs1DForOutWhenUnconnected=off
  wires:
  In1/1 -> Out1/1

== system ASM_Traffic_A11/VehicleDynamics/Interface_Out/Animation/Const_r_unloaded_Tire_FL[m] ==
  In1 : Inport
  Out1 : Outport  VectorParamsAs1DForOutWhenUnconnected=off
  wires:
  In1/1 -> Out1/1

== system ASM_Traffic_A11/VehicleDynamics/Interface_Out/Animation/Const_r_unloaded_Tire_FR[m] ==
  In1 : Inport
  Out1 : Outport  VectorParamsAs1DForOutWhenUnconnected=off
  wires:
  In1/1 -> Out1/1

== system ASM_Traffic_A11/VehicleDynamics/Interface_Out/Animation/Const_r_unloaded_Tire_RL[m] ==
  In1 : Inport
  Out1 : Outport  VectorParamsAs1DForOutWhenUnconnected=off
  wires:
  In1/1 -> Out1/1

== system ASM_Traffic_A11/VehicleDynamics/Interface_Out/Animation/Const_r_unloaded_Tire_RR[m] ==
  In1 : Inport
  Out1 : Outport  VectorParamsAs1DForOutWhenUnconnected=off
  wires:
  In1/1 -> Out1/1

== system ASM_Traffic_A11/VehicleDynamics/Interface_Out/Animation/F_FL_Tire_CoorSys_V[x;y;z][N] ==
  In1 : Inport
  Out1 : Outport  VectorParamsAs1DForOutWhenUnconnected=off
  wires:
  In1/1 -> Out1/1

== system ASM_Traffic_A11/VehicleDynamics/Interface_Out/Animation/F_FR_Tire_CoorSys_V[x;y;z][N] ==
  In1 : Inport
  Out1 : Outport  VectorParamsAs1DForOutWhenUnconnected=off
  wires:
  In1/1 -> Out1/1

== system ASM_Traffic_A11/VehicleDynamics/Interface_Out/Animation/F_RL_Tire_CoorSys_V[x;y;z][N] ==
  In1 : Inport
  Out1 : Outport  VectorParamsAs1DForOutWhenUnconnected=off
  wires:
  In1/1 -> Out1/1

== system ASM_Traffic_A11/VehicleDynamics/Interface_Out/Animation/F_RR_Tire_CoorSys_V[x;y;z][N] ==
  In1 : Inport
  Out1 : Outport  VectorParamsAs1DForOutWhenUnconnected=off
  wires:
  In1/1 -> Out1/1

== system ASM_Traffic_A11/VehicleDynamics/Interface_Out/Animation/Pos_FL_Wheel[x;y;z][m] ==
  In1 : Inport
  Out1 : Outport  VectorParamsAs1DForOutWhenUnconnected=off
  wires:
  In1/1 -> Out1/1

== system ASM_Traffic_A11/VehicleDynamics/Interface_Out/Animation/Pos_FR_Wheel[x;y;z][m] ==
  In1 : Inport
  Out1 : Outport  VectorParamsAs1DForOutWhenUnconnected=off
  wires:
  In1/1 -> Out1/1

== system ASM_Traffic_A11/VehicleDynamics/Interface_Out/Animation/Pos_RL_Wheel[x;y;z][m] ==
  In2 : Inport
  Out2 : Outport  VectorParamsAs1DForOutWhenUnconnected=off
  wires:
  In2/1 -> Out2/1

== system ASM_Traffic_A11/VehicleDynamics/Interface_Out/Animation/Pos_RR_Wheel[x;y;z][m] ==
  In1 : Inport
  Out1 : Outport  VectorParamsAs1DForOutWhenUnconnected=off
  wires:
  In1/1 -> Out1/1

== system ASM_Traffic_A11/VehicleDynamics/Interface_Out/Animation/Pos_Vehicle_CoorSys_E[x;y;z][m] ==
  In1 : Inport
  Out1 : Outport  VectorParamsAs1DForOutWhenUnconnected=off
  wires:
  In1/1 -> Out1/1

== system ASM_Traffic_A11/VehicleDynamics/Interface_Out/Animation/YawRate_Vehicle_CoG[deg|s] ==
  In1 : Inport
  Out1 : Outport  VectorParamsAs1DForOutWhenUnconnected=off
  wires:
  In1/1 -> Out1/1

== system ASM_Traffic_A11/VehicleDynamics/Interface_Out/Animation/a_y_Vehicle_CoG[m|s2] ==
  In1 : Inport
  Out1 : Outport  VectorParamsAs1DForOutWhenUnconnected=off
  wires:
  In1/1 -> Out1/1

== system ASM_Traffic_A11/VehicleDynamics/Interface_Out/Animation/p_Brake[FL;FR;RL;RR][bar] ==
  In1 : Inport
  Out1 : Outport  VectorParamsAs1DForOutWhenUnconnected=off
  wires:
  In1/1 -> Out1/1

== system ASM_Traffic_A11/VehicleDynamics/Interface_Out/Animation/r_Dyn_FL_Tire[m] ==
  In1 : Inport
  Out1 : Outport  VectorParamsAs1DForOutWhenUnconnected=off
  wires:
  In1/1 -> Out1/1

== system ASM_Traffic_A11/VehicleDynamics/Interface_Out/Animation/r_Dyn_FR_Tire[m] ==
  In1 : Inport
  Out1 : Outport  VectorParamsAs1DForOutWhenUnconnected=off
  wires:
  In1/1 -> Out1/1

== system ASM_Traffic_A11/VehicleDynamics/Interface_Out/Animation/r_Dyn_RL_Tire[m] ==
  In1 : Inport
  Out1 : Outport  VectorParamsAs1DForOutWhenUnconnected=off
  wires:
  In1/1 -> Out1/1

== system ASM_Traffic_A11/VehicleDynamics/Interface_Out/Animation/r_Dyn_RR_Tire[m] ==
  In1 : Inport
  Out1 : Outport  VectorParamsAs1DForOutWhenUnconnected=off
  wires:
  In1/1 -> Out1/1

== system ASM_Traffic_A11/VehicleDynamics/Interface_Out/Animation/s_Vehicle[m] ==
  In1 : Inport
  Out1 : Outport  VectorParamsAs1DForOutWhenUnconnected=off
  wires:
  In1/1 -> Out1/1

== system ASM_Traffic_A11/VehicleDynamics/Interface_Out/Animation/v_x_Vehicle_CoG[km|h] ==
  In1 : Inport
  Out1 : Outport  VectorParamsAs1DForOutWhenUnconnected=off
  wires:
  In1/1 -> Out1/1

== system ASM_Traffic_A11/VehicleDynamics/Interface_Out/Control_ModelSignals/ECU_ESP_Mode[0None|1ABS|2ESP|3ASR]_ ==
  In1 : Inport
  Gain : Gain  SaturateOnIntegerOverflow=on  OutDataTypeStr=Inherit: Same as input  ParamDataTypeStr=Inherit: Same as input
  Out1 : Outport  VectorParamsAs1DForOutWhenUnconnected=off
  wires:
  Gain/1 -> Out1/1
  In1/1 -> Gain/1

== system ASM_Traffic_A11/VehicleDynamics/Interface_Out/Control_ModelSignals/Enable_TrqDecrease_Fast_ESP[0|1]_ ==
  In1 : Inport
  Gain : Gain  SaturateOnIntegerOverflow=on  OutDataTypeStr=Inherit: Same as input  ParamDataTypeStr=Inherit: Same as input
  Out1 : Outport  VectorParamsAs1DForOutWhenUnconnected=off
  wires:
  Gain/1 -> Out1/1
  In1/1 -> Gain/1

== system ASM_Traffic_A11/VehicleDynamics/Interface_Out/Control_ModelSignals/Enable_TrqDecrease_Slow_ESP[0|1]_ ==
  In1 : Inport
  Gain : Gain  SaturateOnIntegerOverflow=on  OutDataTypeStr=Inherit: Same as input  ParamDataTypeStr=Inherit: Same as input
  Out1 : Outport  VectorParamsAs1DForOutWhenUnconnected=off
  wires:
  Gain/1 -> Out1/1
  In1/1 -> Gain/1

== system ASM_Traffic_A11/VehicleDynamics/Interface_Out/Control_ModelSignals/Enable_TrqIncrease_ESP[0|1]_ ==
  In1 : Inport
  Gain : Gain  SaturateOnIntegerOverflow=on  OutDataTypeStr=Inherit: Same as input  ParamDataTypeStr=Inherit: Same as input
  Out1 : Outport  VectorParamsAs1DForOutWhenUnconnected=off
  wires:
  Gain/1 -> Out1/1
  In1/1 -> Gain/1

== system ASM_Traffic_A11/VehicleDynamics/Interface_Out/Control_ModelSignals/Enable_p_Brake_Desired[0|1]_ ==
  In1 : Inport
  Gain : Gain  SaturateOnIntegerOverflow=on  OutDataTypeStr=Inherit: Same as input  ParamDataTypeStr=Inherit: Same as input
  Out1 : Outport  VectorParamsAs1DForOutWhenUnconnected=off
  wires:
  Gain/1 -> Out1/1
  In1/1 -> Gain/1

== system ASM_Traffic_A11/VehicleDynamics/Interface_Out/Control_ModelSignals/Trq_DecreaseRequest_Fast_ESP[Nm]_ ==
  In1 : Inport
  Gain : Gain  SaturateOnIntegerOverflow=on  OutDataTypeStr=Inherit: Same as input  ParamDataTypeStr=Inherit: Same as input
  Out1 : Outport  VectorParamsAs1DForOutWhenUnconnected=off
  wires:
  Gain/1 -> Out1/1
  In1/1 -> Gain/1

== system ASM_Traffic_A11/VehicleDynamics/Interface_Out/Control_ModelSignals/Trq_DecreaseRequest_Slow_ESP[Nm]_ ==
  In1 : Inport
  Gain : Gain  SaturateOnIntegerOverflow=on  OutDataTypeStr=Inherit: Same as input  ParamDataTypeStr=Inherit: Same as input
  Out1 : Outport  VectorParamsAs1DForOutWhenUnconnected=off
  wires:
  Gain/1 -> Out1/1
  In1/1 -> Gain/1

== system ASM_Traffic_A11/VehicleDynamics/Interface_Out/Control_ModelSignals/Trq_IncreaseRequest_ESP[Nm]_ ==
  In1 : Inport
  Gain : Gain  SaturateOnIntegerOverflow=on  OutDataTypeStr=Inherit: Same as input  ParamDataTypeStr=Inherit: Same as input
  Out1 : Outport  VectorParamsAs1DForOutWhenUnconnected=off
  wires:
  Gain/1 -> Out1/1
  In1/1 -> Gain/1

== system ASM_Traffic_A11/VehicleDynamics/Interface_Out/Control_ModelSignals/p_Brake_Desired[bar]_ ==
  In1 : Inport
  Gain : Gain  SaturateOnIntegerOverflow=on  OutDataTypeStr=Inherit: Same as input  ParamDataTypeStr=Inherit: Same as input
  Out1 : Outport  VectorParamsAs1DForOutWhenUnconnected=off
  wires:
  Gain/1 -> Out1/1
  In1/1 -> Gain/1

== system ASM_Traffic_A11/VehicleDynamics/Interface_Out/Plant_ModelSignals/Active_CP_VehDyn[]_ ==
  In1 : Inport
  Gain : Gain  SaturateOnIntegerOverflow=on  OutDataTypeStr=Inherit: Same as input  ParamDataTypeStr=Inherit: Same as input
  Out1 : Outport  VectorParamsAs1DForOutWhenUnconnected=off
  wires:
  In1/1 -> Gain/1
  Gain/1 -> Out1/1

== system ASM_Traffic_A11/VehicleDynamics/Interface_Out/Plant_ModelSignals/Angle_SteeringWheel[deg]_ ==
  In1 : Inport
  Gain : Gain  SaturateOnIntegerOverflow=on  OutDataTypeStr=Inherit: Same as input  ParamDataTypeStr=Inherit: Same as input
  Out1 : Outport  VectorParamsAs1DForOutWhenUnconnected=off
  wires:
  Gain/1 -> Out1/1
  In1/1 -> Gain/1

== system ASM_Traffic_A11/VehicleDynamics/Interface_Out/Plant_ModelSignals/Angle_SteeringWheel_dt[deg|s]_ ==
  In1 : Inport
  Gain : Gain  SaturateOnIntegerOverflow=on  OutDataTypeStr=Inherit: Same as input  ParamDataTypeStr=Inherit: Same as input
  Out1 : Outport  VectorParamsAs1DForOutWhenUnconnected=off
  wires:
  Gain/1 -> Out1/1
  In1/1 -> Gain/1

== system ASM_Traffic_A11/VehicleDynamics/Interface_Out/Plant_ModelSignals/Angle_Vehicle_CoorSys_E[x;y;z][deg]_ ==
  In1 : Inport
  Gain : Gain  SaturateOnIntegerOverflow=on  OutDataTypeStr=Inherit: Same as input  ParamDataTypeStr=Inherit: Same as input
  Out1 : Outport  VectorParamsAs1DForOutWhenUnconnected=off
  wires:
  Gain/1 -> Out1/1
  In1/1 -> Gain/1

== system ASM_Traffic_A11/VehicleDynamics/Interface_Out/Plant_ModelSignals/Angle_Yaw_Vehicle_CoorSys_E[deg]_ ==
  In1 : Inport
  Gain : Gain  SaturateOnIntegerOverflow=on  OutDataTypeStr=Inherit: Same as input  ParamDataTypeStr=Inherit: Same as input
  Out1 : Outport  VectorParamsAs1DForOutWhenUnconnected=off
  wires:
  In1/1 -> Gain/1
  Gain/1 -> Out1/1

== system ASM_Traffic_A11/VehicleDynamics/Interface_Out/Plant_ModelSignals/Coef_RollingRes[FL;FR;RL;RR][]_ ==
  In1 : Inport
  Gain : Gain  SaturateOnIntegerOverflow=on  OutDataTypeStr=Inherit: Same as input  ParamDataTypeStr=Inherit: Same as input
  Out1 : Outport  VectorParamsAs1DForOutWhenUnconnected=off
  wires:
  Gain/1 -> Out1/1
  In1/1 -> Gain/1

== system ASM_Traffic_A11/VehicleDynamics/Interface_Out/Plant_ModelSignals/Coef_RollingRes_Mean[]_ ==
  In1 : Inport
  Gain : Gain  SaturateOnIntegerOverflow=on  OutDataTypeStr=Inherit: Same as input  ParamDataTypeStr=Inherit: Same as input
  Out1 : Outport  VectorParamsAs1DForOutWhenUnconnected=off
  wires:
  Gain/1 -> Out1/1
  In1/1 -> Gain/1

== system ASM_Traffic_A11/VehicleDynamics/Interface_Out/Plant_ModelSignals/Const_r_unloaded_Tire_Mean[m]_ ==
  In1 : Inport
  Gain : Gain  SaturateOnIntegerOverflow=on  OutDataTypeStr=Inherit: Same as input  ParamDataTypeStr=Inherit: Same as input
  Out1 : Outport  VectorParamsAs1DForOutWhenUnconnected=off
  wires:
  Gain/1 -> Out1/1
  In1/1 -> Gain/1

== system ASM_Traffic_A11/VehicleDynamics/Interface_Out/Plant_ModelSignals/CorneringStiffness[FL;FR;RL;RR][N]_ ==
  In1 : Inport
  Gain : Gain  SaturateOnIntegerOverflow=on  OutDataTypeStr=Inherit: Same as input  ParamDataTypeStr=Inherit: Same as input
  Out1 : Outport  VectorParamsAs1DForOutWhenUnconnected=off
  wires:
  Gain/1 -> Out1/1
  In1/1 -> Gain/1

== system ASM_Traffic_A11/VehicleDynamics/Interface_Out/Plant_ModelSignals/CorneringStiffness_Tire_Front[N|rad]_ ==
  In1 : Inport
  Gain : Gain  SaturateOnIntegerOverflow=on  OutDataTypeStr=Inherit: Same as input  ParamDataTypeStr=Inherit: Same as input
  Out1 : Outport  VectorParamsAs1DForOutWhenUnconnected=off
  wires:
  Gain/1 -> Out1/1
  In1/1 -> Gain/1

== system ASM_Traffic_A11/VehicleDynamics/Interface_Out/Plant_ModelSignals/CorneringStiffness_Tire_Rear[N|rad]_ ==
  In1 : Inport
  Gain : Gain  SaturateOnIntegerOverflow=on  OutDataTypeStr=Inherit: Same as input  ParamDataTypeStr=Inherit: Same as input
  Out1 : Outport  VectorParamsAs1DForOutWhenUnconnected=off
  wires:
  In1/1 -> Gain/1
  Gain/1 -> Out1/1

== system ASM_Traffic_A11/VehicleDynamics/Interface_Out/Plant_ModelSignals/Cw_x[]_ ==
  In1 : Inport
  Gain : Gain  SaturateOnIntegerOverflow=on  OutDataTypeStr=Inherit: Same as input  ParamDataTypeStr=Inherit: Same as input
  Out1 : Outport  VectorParamsAs1DForOutWhenUnconnected=off
  wires:
  Gain/1 -> Out1/1
  In1/1 -> Gain/1

== system ASM_Traffic_A11/VehicleDynamics/Interface_Out/Plant_ModelSignals/F_Driving_Res[N]_ ==
  In1 : Inport
  Gain : Gain  SaturateOnIntegerOverflow=on  OutDataTypeStr=Inherit: Same as input  ParamDataTypeStr=Inherit: Same as input
  Out1 : Outport  VectorParamsAs1DForOutWhenUnconnected=off
  wires:
  Gain/1 -> Out1/1
  In1/1 -> Gain/1

== system ASM_Traffic_A11/VehicleDynamics/Interface_Out/Plant_ModelSignals/F_Vehicle_Gravitational[x;y;z][N]_ ==
  In1 : Inport
  Gain : Gain  SaturateOnIntegerOverflow=on  OutDataTypeStr=Inherit: Same as input  ParamDataTypeStr=Inherit: Same as input
  Out1 : Outport  VectorParamsAs1DForOutWhenUnconnected=off
  wires:
  Gain/1 -> Out1/1
  In1/1 -> Gain/1

== system ASM_Traffic_A11/VehicleDynamics/Interface_Out/Plant_ModelSignals/F_x_Aero_CoorSys_V[N]_ ==
  In1 : Inport
  Gain : Gain  SaturateOnIntegerOverflow=on  OutDataTypeStr=Inherit: Same as input  ParamDataTypeStr=Inherit: Same as input
  Out1 : Outport  VectorParamsAs1DForOutWhenUnconnected=off
  wires:
  Gain/1 -> Out1/1
  In1/1 -> Gain/1

== system ASM_Traffic_A11/VehicleDynamics/Interface_Out/Plant_ModelSignals/Inertia_z_Vehicle_Total[kgm2]_ ==
  In1 : Inport
  Gain : Gain  SaturateOnIntegerOverflow=on  OutDataTypeStr=Inherit: Same as input  ParamDataTypeStr=Inherit: Same as input
  Out1 : Outport  VectorParamsAs1DForOutWhenUnconnected=off
  wires:
  Gain/1 -> Out1/1
  In1/1 -> Gain/1

== system ASM_Traffic_A11/VehicleDynamics/Interface_Out/Plant_ModelSignals/PitchRate_Vehicle_CoG[deg|s]_ ==
  In1 : Inport
  Gain : Gain  SaturateOnIntegerOverflow=on  OutDataTypeStr=Inherit: Same as input  ParamDataTypeStr=Inherit: Same as input
  Out1 : Outport  VectorParamsAs1DForOutWhenUnconnected=off
  wires:
  Gain/1 -> Out1/1
  In1/1 -> Gain/1

== system ASM_Traffic_A11/VehicleDynamics/Interface_Out/Plant_ModelSignals/Pos_CP_FL_CoorSys_E[x;y][m]_ ==
  In1 : Inport
  Gain : Gain  SaturateOnIntegerOverflow=on  OutDataTypeStr=Inherit: Same as input  ParamDataTypeStr=Inherit: Same as input
  Out1 : Outport  VectorParamsAs1DForOutWhenUnconnected=off
  wires:
  Gain/1 -> Out1/1
  In1/1 -> Gain/1

== system ASM_Traffic_A11/VehicleDynamics/Interface_Out/Plant_ModelSignals/Pos_CP_FR_CoorSys_E[x;y][m]_ ==
  In1 : Inport
  Gain : Gain  SaturateOnIntegerOverflow=on  OutDataTypeStr=Inherit: Same as input  ParamDataTypeStr=Inherit: Same as input
  Out1 : Outport  VectorParamsAs1DForOutWhenUnconnected=off
  wires:
  Gain/1 -> Out1/1
  In1/1 -> Gain/1

== system ASM_Traffic_A11/VehicleDynamics/Interface_Out/Plant_ModelSignals/Pos_CP_Front_CoorSys_E[x;y][m]_ ==
  In1 : Inport
  Gain : Gain  SaturateOnIntegerOverflow=on  OutDataTypeStr=Inherit: Same as input  ParamDataTypeStr=Inherit: Same as input
  Out1 : Outport  VectorParamsAs1DForOutWhenUnconnected=off
  wires:
  In1/1 -> Gain/1
  Gain/1 -> Out1/1

== system ASM_Traffic_A11/VehicleDynamics/Interface_Out/Plant_ModelSignals/Pos_CP_R2L2_CoorSys_E[x;y][m]_ ==
  In1 : Inport
  Gain : Gain  SaturateOnIntegerOverflow=on  OutDataTypeStr=Inherit: Same as input  ParamDataTypeStr=Inherit: Same as input
  Out1 : Outport  VectorParamsAs1DForOutWhenUnconnected=off
  wires:
  Gain/1 -> Out1/1
  In1/1 -> Gain/1

== system ASM_Traffic_A11/VehicleDynamics/Interface_Out/Plant_ModelSignals/Pos_CP_R2L_CoorSys_E[x;y][m]_ ==
  In1 : Inport
  Gain : Gain  SaturateOnIntegerOverflow=on  OutDataTypeStr=Inherit: Same as input  ParamDataTypeStr=Inherit: Same as input
  Out1 : Outport  VectorParamsAs1DForOutWhenUnconnected=off
  wires:
  Gain/1 -> Out1/1
  In1/1 -> Gain/1

== system ASM_Traffic_A11/VehicleDynamics/Interface_Out/Plant_ModelSignals/Pos_CP_R2R2_CoorSys_E[x;y][m]_ ==
  In1 : Inport
  Gain : Gain  SaturateOnIntegerOverflow=on  OutDataTypeStr=Inherit: Same as input  ParamDataTypeStr=Inherit: Same as input
  Out1 : Outport  VectorParamsAs1DForOutWhenUnconnected=off
  wires:
  Gain/1 -> Out1/1
  In1/1 -> Gain/1

== system ASM_Traffic_A11/VehicleDynamics/Interface_Out/Plant_ModelSignals/Pos_CP_R2R_CoorSys_E[x;y][m]_ ==
  In1 : Inport
  Gain : Gain  SaturateOnIntegerOverflow=on  OutDataTypeStr=Inherit: Same as input  ParamDataTypeStr=Inherit: Same as input
  Out1 : Outport  VectorParamsAs1DForOutWhenUnconnected=off
  wires:
  Gain/1 -> Out1/1
  In1/1 -> Gain/1

== system ASM_Traffic_A11/VehicleDynamics/Interface_Out/Plant_ModelSignals/Pos_CP_RL2_CoorSys_E[x;y][m]_ ==
  In1 : Inport
  Gain : Gain  SaturateOnIntegerOverflow=on  OutDataTypeStr=Inherit: Same as input  ParamDataTypeStr=Inherit: Same as input
  Out1 : Outport  VectorParamsAs1DForOutWhenUnconnected=off
  wires:
  Gain/1 -> Out1/1
  In1/1 -> Gain/1

== system ASM_Traffic_A11/VehicleDynamics/Interface_Out/Plant_ModelSignals/Pos_CP_RL_CoorSys_E[x;y][m]_ ==
  In1 : Inport
  Gain : Gain  SaturateOnIntegerOverflow=on  OutDataTypeStr=Inherit: Same as input  ParamDataTypeStr=Inherit: Same as input
  Out1 : Outport  VectorParamsAs1DForOutWhenUnconnected=off
  wires:
  Gain/1 -> Out1/1
  In1/1 -> Gain/1

== system ASM_Traffic_A11/VehicleDynamics/Interface_Out/Plant_ModelSignals/Pos_CP_RR2_CoorSys_E[x;y][m]_ ==
  In1 : Inport
  Gain : Gain  SaturateOnIntegerOverflow=on  OutDataTypeStr=Inherit: Same as input  ParamDataTypeStr=Inherit: Same as input
  Out1 : Outport  VectorParamsAs1DForOutWhenUnconnected=off
  wires:
  Gain/1 -> Out1/1
  In1/1 -> Gain/1

== system ASM_Traffic_A11/VehicleDynamics/Interface_Out/Plant_ModelSignals/Pos_CP_RR_CoorSys_E[x;y][m]_ ==
  In1 : Inport
  Gain : Gain  SaturateOnIntegerOverflow=on  OutDataTypeStr=Inherit: Same as input  ParamDataTypeStr=Inherit: Same as input
  Out1 : Outport  VectorParamsAs1DForOutWhenUnconnected=off
  wires:
  Gain/1 -> Out1/1
  In1/1 -> Gain/1

== system ASM_Traffic_A11/VehicleDynamics/Interface_Out/Plant_ModelSignals/Pos_CP_Rear_CoorSys_E[x;y][m]_ ==
  In1 : Inport
  Gain : Gain  SaturateOnIntegerOverflow=on  OutDataTypeStr=Inherit: Same as input  ParamDataTypeStr=Inherit: Same as input
  Out1 : Outport  VectorParamsAs1DForOutWhenUnconnected=off
  wires:
  In1/1 -> Gain/1
  Gain/1 -> Out1/1

== system ASM_Traffic_A11/VehicleDynamics/Interface_Out/Plant_ModelSignals/Pos_FL_Wheel[x;y;z][m]_ ==
  In1 : Inport
  Gain : Gain  SaturateOnIntegerOverflow=on  OutDataTypeStr=Inherit: Same as input  ParamDataTypeStr=Inherit: Same as input
  Out1 : Outport  VectorParamsAs1DForOutWhenUnconnected=off
  wires:
  Gain/1 -> Out1/1
  In1/1 -> Gain/1

== system ASM_Traffic_A11/VehicleDynamics/Interface_Out/Plant_ModelSignals/Pos_FR_Wheel[x;y;z][m]_ ==
  In1 : Inport
  Gain : Gain  SaturateOnIntegerOverflow=on  OutDataTypeStr=Inherit: Same as input  ParamDataTypeStr=Inherit: Same as input
  Out1 : Outport  VectorParamsAs1DForOutWhenUnconnected=off
  wires:
  Gain/1 -> Out1/1
  In1/1 -> Gain/1

== system ASM_Traffic_A11/VehicleDynamics/Interface_Out/Plant_ModelSignals/Pos_RL_Wheel[x;y;z][m]_ ==
  In1 : Inport
  Gain : Gain  SaturateOnIntegerOverflow=on  OutDataTypeStr=Inherit: Same as input  ParamDataTypeStr=Inherit: Same as input
  Out1 : Outport  VectorParamsAs1DForOutWhenUnconnected=off
  wires:
  Gain/1 -> Out1/1
  In1/1 -> Gain/1

== system ASM_Traffic_A11/VehicleDynamics/Interface_Out/Plant_ModelSignals/Pos_RR_Wheel[x;y;z][m]_ ==
  In1 : Inport
  Gain : Gain  SaturateOnIntegerOverflow=on  OutDataTypeStr=Inherit: Same as input  ParamDataTypeStr=Inherit: Same as input
  Out1 : Outport  VectorParamsAs1DForOutWhenUnconnected=off
  wires:
  Gain/1 -> Out1/1
  In1/1 -> Gain/1

== system ASM_Traffic_A11/VehicleDynamics/Interface_Out/Plant_ModelSignals/Pos_Vehicle_CoorSys_E[x;y;z][m]_ ==
  In1 : Inport
  Gain : Gain  SaturateOnIntegerOverflow=on  OutDataTypeStr=Inherit: Same as input  ParamDataTypeStr=Inherit: Same as input
  Out1 : Outport  VectorParamsAs1DForOutWhenUnconnected=off
  wires:
  Gain/1 -> Out1/1
  In1/1 -> Gain/1

== system ASM_Traffic_A11/VehicleDynamics/Interface_Out/Plant_ModelSignals/Pos_x_CoG_Vehicle_Total[m]_ ==
  In1 : Inport
  Gain : Gain  SaturateOnIntegerOverflow=on  OutDataTypeStr=Inherit: Same as input  ParamDataTypeStr=Inherit: Same as input
  Out1 : Outport  VectorParamsAs1DForOutWhenUnconnected=off
  wires:
  Gain/1 -> Out1/1
  In1/1 -> Gain/1

== system ASM_Traffic_A11/VehicleDynamics/Interface_Out/Plant_ModelSignals/Pos_x_Vehicle_CoorSys_E[m]_ ==
  In1 : Inport
  Gain : Gain  SaturateOnIntegerOverflow=on  OutDataTypeStr=Inherit: Same as input  ParamDataTypeStr=Inherit: Same as input
  Out1 : Outport  VectorParamsAs1DForOutWhenUnconnected=off
  wires:
  In1/1 -> Gain/1
  Gain/1 -> Out1/1

== system ASM_Traffic_A11/VehicleDynamics/Interface_Out/Plant_ModelSignals/Pos_y_Vehicle_CoorSys_E[m]_ ==
  In1 : Inport
  Gain : Gain  SaturateOnIntegerOverflow=on  OutDataTypeStr=Inherit: Same as input  ParamDataTypeStr=Inherit: Same as input
  Out1 : Outport  VectorParamsAs1DForOutWhenUnconnected=off
  wires:
  Gain/1 -> Out1/1
  In1/1 -> Gain/1

== system ASM_Traffic_A11/VehicleDynamics/Interface_Out/Plant_ModelSignals/RollRate_Vehicle_CoG[deg|s]_ ==
  In1 : Inport
  Gain : Gain  SaturateOnIntegerOverflow=on  OutDataTypeStr=Inherit: Same as input  ParamDataTypeStr=Inherit: Same as input
  Out1 : Outport  VectorParamsAs1DForOutWhenUnconnected=off
  wires:
  Gain/1 -> Out1/1
  In1/1 -> Gain/1

== system ASM_Traffic_A11/VehicleDynamics/Interface_Out/Plant_ModelSignals/RotationMatrix_V_to_E[1x9]_ ==
  In1 : Inport
  Gain : Gain  SaturateOnIntegerOverflow=on  OutDataTypeStr=Inherit: Same as input  ParamDataTypeStr=Inherit: Same as input
  Out1 : Outport  VectorParamsAs1DForOutWhenUnconnected=off
  wires:
  Gain/1 -> Out1/1
  In1/1 -> Gain/1

== system ASM_Traffic_A11/VehicleDynamics/Interface_Out/Plant_ModelSignals/RotationMatrix_V_to_E_T[1x9]_ ==
  In1 : Inport
  Gain : Gain  SaturateOnIntegerOverflow=on  OutDataTypeStr=Inherit: Same as input  ParamDataTypeStr=Inherit: Same as input
  Out1 : Outport  VectorParamsAs1DForOutWhenUnconnected=off
  wires:
  Gain/1 -> Out1/1
  In1/1 -> Gain/1

== system ASM_Traffic_A11/VehicleDynamics/Interface_Out/Plant_ModelSignals/Slip_x_Wheel[]_ ==
  In1 : Inport
  Gain : Gain  SaturateOnIntegerOverflow=on  OutDataTypeStr=Inherit: Same as input  ParamDataTypeStr=Inherit: Same as input
  Out1 : Outport  VectorParamsAs1DForOutWhenUnconnected=off
  wires:
  In1/1 -> Gain/1
  Gain/1 -> Out1/1

== system ASM_Traffic_A11/VehicleDynamics/Interface_Out/Plant_ModelSignals/Sw_MasterBrakeCylinder_Mode[1linear|2physical|3Booster]_ ==
  In1 : Inport
  Gain : Gain  SaturateOnIntegerOverflow=on  OutDataTypeStr=Inherit: Same as input  ParamDataTypeStr=Inherit: Same as input
  Out1 : Outport  VectorParamsAs1DForOutWhenUnconnected=off
  wires:
  Gain/1 -> Out1/1
  In1/1 -> Gain/1

== system ASM_Traffic_A11/VehicleDynamics/Interface_Out/Plant_ModelSignals/Sw_Rotation[1Cardan|2ToeCamberCaster]_ ==
  In1 : Inport
  Gain : Gain  SaturateOnIntegerOverflow=on  OutDataTypeStr=Inherit: Same as input  ParamDataTypeStr=Inherit: Same as input
  Out1 : Outport  VectorParamsAs1DForOutWhenUnconnected=off
  wires:
  Gain/1 -> Out1/1
  In1/1 -> Gain/1

== system ASM_Traffic_A11/VehicleDynamics/Interface_Out/Plant_ModelSignals/Sw_r_Tire[1:intern;2:extern]_ ==
  In1 : Inport
  Gain : Gain  SaturateOnIntegerOverflow=on  OutDataTypeStr=Inherit: Same as input  ParamDataTypeStr=Inherit: Same as input
  Out1 : Outport  VectorParamsAs1DForOutWhenUnconnected=off
  wires:
  In1/1 -> Gain/1
  Gain/1 -> Out1/1

== system ASM_Traffic_A11/VehicleDynamics/Interface_Out/Plant_ModelSignals/Trq_Max_Brake[Nm]_ ==
  In1 : Inport
  Gain : Gain  SaturateOnIntegerOverflow=on  OutDataTypeStr=Inherit: Same as input  ParamDataTypeStr=Inherit: Same as input
  Out1 : Outport  VectorParamsAs1DForOutWhenUnconnected=off
  wires:
  Gain/1 -> Out1/1
  In1/1 -> Gain/1
